simulink model "ADRC_PTAR_ALL"  (R2025b)
settings: Solver=VariableStepAuto  StartTime=0.0  StopTime=500000  RelTol=1e-3
undefined symbols (not defined in the file): a0, a1, a2, a3, a4, a5, A_o, b0, Bau, E1, K, k, L, L_E, m, P_, Tau
libraries: slpidlib x1
settings Model: Creator=esteban  LastModifiedBy=esteban

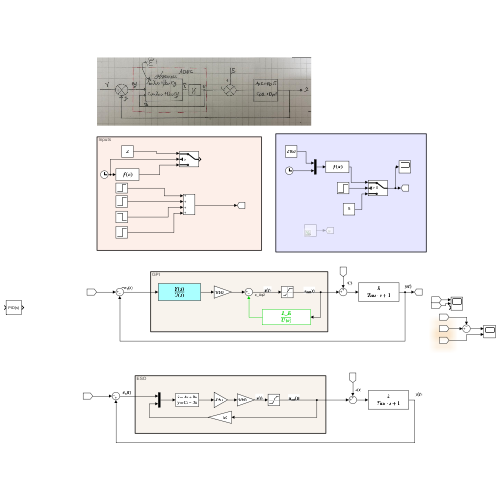
[thumbnail: Simulink's stored preview of the top-level diagram]
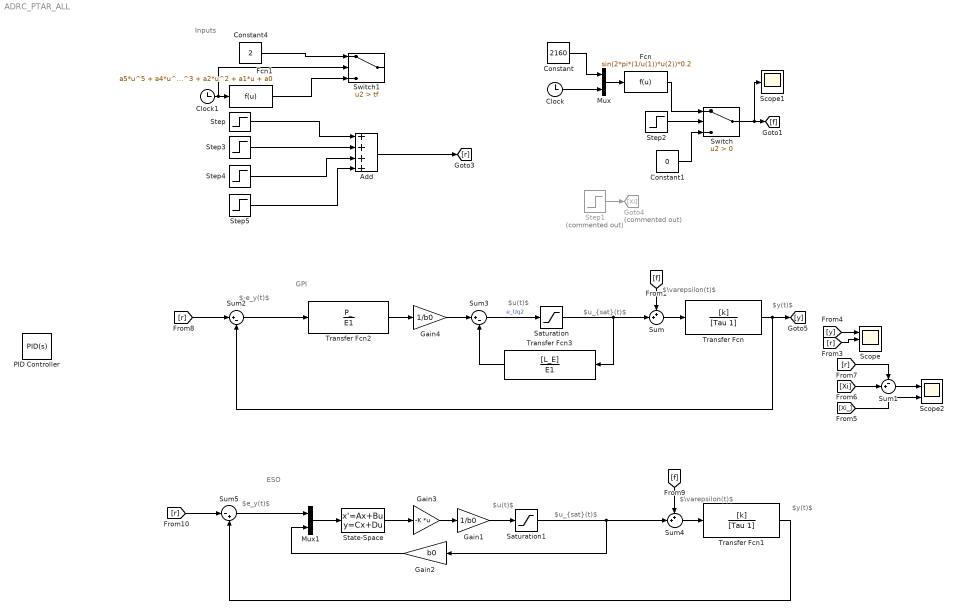
== system ADRC_PTAR_ALL ==
  note: Inputs
  note: GPI
  note: $y(t)$
  note: $u_{sat}(t)$
  note: $u(t)$
  note: $-e_y(t)$
  note: $u(t)$
  note: $u_{sat}(t)$
  note: $y(t)$
  note: $e_y(t)$
  note: ESO
  note: $\varepsilon(t)$
  note: $\varepsilon(t)$
  Add : Sum  Inputs=++++
  Clock : Clock
  Clock1 : Clock
  Constant : Constant  Value=2160
  Constant1 : Constant  Value=0
  Constant4 : Constant  Value=2
  Fcn : Fcn  Expr=sin(2*pi*(1/u(1))*u(2))*0.2
  Fcn1 : Fcn  Expr=a5*u^5 + a4*u^4 + a3*u^3 + a2*u^2 + a1*u + a0
  Gain1 : Gain  Gain=1/b0
  Gain2 : Gain  Gain=b0
  Gain3 : Gain  Gain=-K  Multiplication=Matrix(K*u)
  Gain4 : Gain  Gain=1/b0
  Goto4 : Goto  Commented=on  GotoTag=Xi
  Mux : Mux  Inputs=2
  Mux1 : Mux  Inputs=2
  PID Controller : slpidlib/PID Controller  Controller=PID  Form=Parallel  TimeDomain=Continuous-time  UseExternalTs=off  SampleTime=-1  IntegratorMethod=Forward Euler  FilterMethod=Forward Euler  ControllerParametersSource=internal  P=1  I=1  UseKiTs=off  D=0  UseExternalDerivativeSource=off  N=100  UseFilter=on  TunerSelectOption=Transfer Function Based (PID Tuner App)  InitialConditionSource=internal  InitialConditionForIntegrator=0  InitialConditionForFilter=0  DifferentiatorICPrevScaledInput=0  ExternalReset=none  TrackingMode=off  Kt=1  LimitOutput=off  SatLimitsSource=internal  UpperSaturationLimit=inf  LowerSaturationLimit=-inf  LinearizeAsGain=on  AntiWindupMode=none  Kb=1  LimitIntegrator=off  UpperIntegratorSaturationLimit=inf  LowerIntegratorSaturationLimit=-inf  POutMin=[]  POutMax=[]  IOutMin=[]  IOutMax=[]  DOutMin=[]  DOutMax=[]  NOutMin=[]  NOutMax=[]  SumOutMin=[]  SumOutMax=[]  SaturationOutMin=[]  SaturationOutMax=[]  PParamMin=[]  PParamMax=[]  IParamMin=[]  IParamMax=[]  DParamMin=[]  DParamMax=[]  NParamMin=[]  NParamMax=[]  KbParamMin=[]  KbParamMax=[]  KtParamMin=[]  KtParamMax=[]  KbOutMin=[]  KbOutMax=[]  KtOutMin=[]  KtOutMax=[]  IntegratorOutMin=[]  IntegratorOutMax=[]  FilterOutMin=[]  FilterOutMax=[]  SumI1OutMin=[]  SumI1OutMax=[]  SumI2OutMin=[]  SumI2OutMax=[]  SumI3OutMin=[]  SumI3OutMax=[]  SumI4OutMin=[]  SumI4OutMax=[]  SumDOutMin=[]  SumDOutMax=[]  DifferentiatorOutMin=[]  DifferentiatorOutMax=[]  FilterDiffOutCoefMin=[]  FilterDiffOutCoefMax=[]  ReciprocalOutMin=[]  ReciprocalOutMax=[]  SumDenOutMin=[]  SumDenOutMax=[]  SumNumOutMin=[]  SumNumOutMax=[]  DivideOutMin=[]  DivideOutMax=[]  UdiffTsProdOutMin=[]  UdiffTsProdOutMax=[]  NTsProdOutMin=[]  NTsProdOutMax=[]  UintegralTsProdOutMin=[]  UintegralTsProdOutMax=[]  UngainTsProdOutMin=[]  UngainTsProdOutMax=[]  ClampingZeroOutDataTypeStr=Inherit: Inherit via back propagation  ClampingZeroOutMin=[]  ClampingZeroOutMax=[]  FilterDenConstantOutDataTypeStr=Inherit: Inherit via back propagation  FilterDenConstantOutMin=[]  FilterDenConstantOutMax=[]  PCopyOutDataTypeStr=Inherit: Inherit via back propagation  PCopyOutMin=[]  PCopyOutMax=[]  NCopyOutDataTypeStr=Inherit: Inherit via back propagation  NCopyOutMin=[]  NCopyOutMax=[]  IntegratorContinuousStateAttributes=''  IntegratorStateMustResolveToSignalObject=off  IntegratorRTWStateStorageClass=Auto  FilterContinuousStateAttributes=''  FilterStateMustResolveToSignalObject=off  FilterRTWStateStorageClass=Auto  ParallelPVariant=InternalParameters  IdealPVariant=Disabled  IVariant=InternalParameters  DVariant=InternalParameters  IntegratorVariant=Continuous  SatVariant=Disabled  AWVariant=Passthrough  PCopyVariant=Disabled  TRVariant=Disabled  FdbkBlocksVariant=Forward  IdealPFdbkVariant=Disabled  SatFdbkVariant=Disabled  DerivativeFilterVariant=ContFilter  NVariant=InternalParameters  NCopyVariant=Disabled  FilterICVariant=InternalICsFilter  IntegratorICVariant=InternalICs  ExternalResetVariant=Disabled  TRSumVariant=Passthrough  SumFdbkVariant=Disabled  SumVariant=Sum_PID  TsampFilterVariant=InternalTs  TsampNgainVariant=Passthrough  TsampIntegralVariant=Disabled_SignalSpec  ExternalSaturationOutDataTypeStr=Inherit: Same as second input  DerivativeSourceVariant=ErrorSignal  PreIntVariant=InternalPreInt
  Saturation : Saturate  UpperLimit=100  LowerLimit=0
  Saturation1 : Saturate  UpperLimit=100  LowerLimit=0
  Scope : Scope  NumInputPorts=3
      settings: ActiveDisplayYMinimum=-0.62844211028159991  ActiveDisplayYMaximum=5.6284389476366234
  Scope1 : Scope
      settings: ActiveDisplayYMinimum=-0.024830958943548569  ActiveDisplayYMaximum=0.2234786304919372  DataLoggingVariableName=ScopeData2
  Scope2 : Scope  NumInputPorts=2
      settings: ActiveDisplayYMinimum=-2.2923205992555511  ActiveDisplayYMaximum=4.2391627723615954  DataLoggingVariableName=ScopeData3
  State-Space : StateSpace  A=A_o  B=[L Bau]  C=eye(m)  D=zeros(m,2)  InitialCondition=0
  Step : Step  Time=40000  After=2  SampleTime=0
  Step1 : Step  Commented=on  Time=4000  After=0.1  SampleTime=0
  Step2 : Step  Time=4000  SampleTime=0
  Step3 : Step  Time=80000  After=0.4  SampleTime=0
  Step4 : Step  Time=120000  After=-0.9  SampleTime=0
  Step5 : Step  Time=160000  After=0.5  SampleTime=0
  Sum : Sum  Inputs=++|
  Sum1 : Sum  Inputs=-+|
  Sum2 : Sum  Inputs=|+-
  Sum3 : Sum  Inputs=|+-
  Sum4 : Sum  Inputs=++|
  Sum5 : Sum  Inputs=|-+
  Switch : Switch  Criteria=u2 > Threshold  SaturateOnIntegerOverflow=off  InputSameDT=off
  Switch1 : Switch  Criteria=u2 > Threshold  Threshold=tf  SaturateOnIntegerOverflow=off  InputSameDT=off
  Transfer Fcn : TransferFcn  Numerator=[k]  Denominator=[Tau 1]
  Transfer Fcn1 : TransferFcn  Numerator=[k]  Denominator=[Tau 1]
  Transfer Fcn2 : TransferFcn  Numerator=P_  Denominator=E1
  Transfer Fcn3 : TransferFcn  Numerator=[L_E]  Denominator=E1
  wires:
  Mux/1 -> Fcn/1
  Clock/1 -> Mux/2
  Constant/1 -> Mux/1
  Step1/1 -> Goto4/1
  Constant1/1 -> Switch/3
  Fcn/1 -> Switch/1
  Step2/1 -> Switch/2
  Switch/1 -> Scope1/1, [f]
  [r] -> Scope/2
  [y] -> Scope/1
  [Xi_] -> Scope2/2
  Sum1/1 -> Scope2/1
  [r] -> Sum1/1
  Step/1 -> Add/1
  Step3/1 -> Add/2
  Step4/1 -> Add/3
  Step5/1 -> Add/4
  [Xi] -> Sum1/2
  Constant4/1 -> Switch1/1
  Clock1/1 -> Switch1/2, Fcn1/1
  Fcn1/1 -> Switch1/3
  Add/1 -> [r]
  [f] -> Sum/1
  Transfer Fcn3/1 -> Sum3/2
  Saturation/1 -> Sum/2, Transfer Fcn3/1
  Sum3/1 -> Saturation/1  "e_Uq2"
  [r] -> Sum2/1
  Sum/1 -> Transfer Fcn/1
  Transfer Fcn/1 -> [y], Sum2/2
  State-Space/1 -> Gain3/1
  Mux1/1 -> State-Space/1
  [r] -> Sum5/1
  Gain1/1 -> Saturation1/1
  [f] -> Sum4/1
  Transfer Fcn1/1 -> Sum5/2
  Sum4/1 -> Transfer Fcn1/1
  Gain3/1 -> Gain1/1
  Sum5/1 -> Mux1/1
  Gain2/1 -> Mux1/2
  Gain4/1 -> Sum3/1
  Transfer Fcn2/1 -> Gain4/1
  Sum2/1 -> Transfer Fcn2/1
  Saturation1/1 -> Sum4/2, Gain2/1
